simulink model "nonlinearAirframe"  (R2026a)
settings: Solver=ode3  StartTime=0  FixedStep=Ts  EnableMultiTasking=on
undefined symbols (not defined in the file): init, Vehicle
libraries: shared6dof x1, aerolibasang x1, dynamicsLibrary x1
settings Model: Creator=The MathWorks, Inc.  LastModifiedBy=khade
settings OptimizationCC: BufferReuse=off
settings DebuggingCC: ParameterPrecisionLossMsg=none
settings HardwareCC: ProdHWDeviceType=32-bit Generic

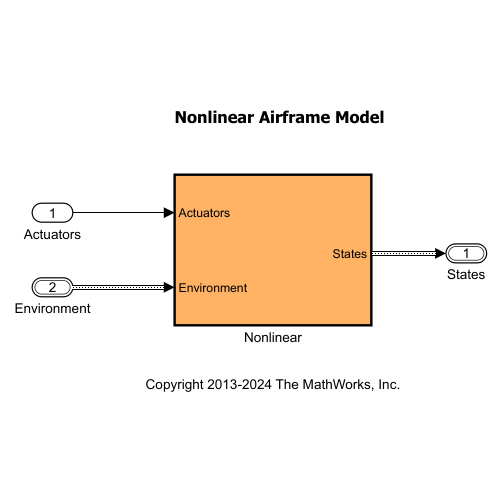
[thumbnail: Simulink's stored preview of the top-level diagram]
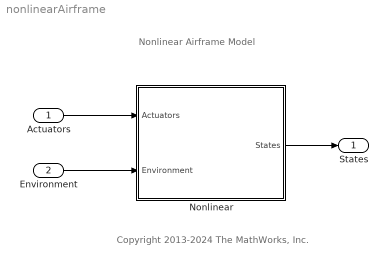
== system nonlinearAirframe ==
  note: Copyright 2013-2024 The MathWorks, Inc.
  note: Nonlinear Airframe Model
  Actuators : Inport  OutDataTypeStr=single  Unit=rpm  PortDimensions=[1 4]
  Environment : Inport  Port=2  OutDataTypeStr=Bus: EnvironmentBus  BusOutputAsStruct=on
  Nonlinear : Subsystem  TreatAsAtomicUnit=on
  States : Outport  OutDataTypeStr=Bus: StatesBus  VectorParamsAs1DForOutWhenUnconnected=off  BusOutputAsStruct=on
  wires:
  Actuators/1 -> Nonlinear/1(Actuators)
  Environment/1 -> Nonlinear/2(Environment)
  Nonlinear/1(States) -> States/1

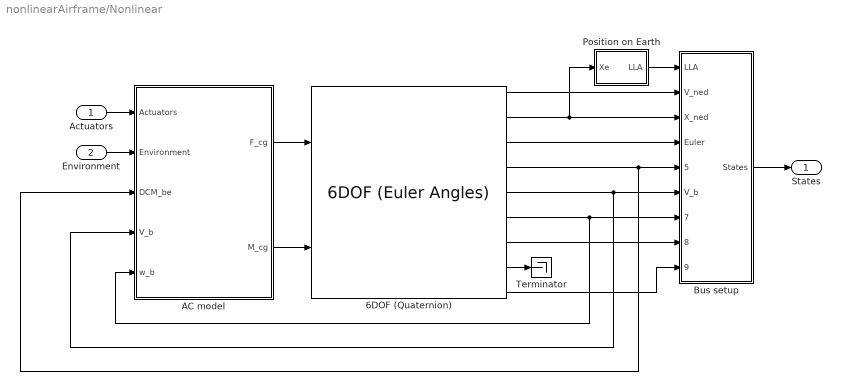
== system nonlinearAirframe/Nonlinear ==
  Actuators : Inport
  Environment : Inport  Port=2
  6DOF (Quaternion) : shared6dof/6DOF (Euler Angles)  units=Metric (MKS)  mtype=Fixed  rep=Euler Angles  xme_0=init.posNED  Vm_0=init.vb  eul_0=init.euler  pm_0=init.angRates  mass_0=Vehicle.Airframe.mass  mass_e=0.5  mass_f=2.0  inertia=Vehicle.Airframe.inertia  inertia_e=eye(3)  inertia_f=2*eye(3)  k_quat=Vehicle.SixDOF.quatGain  vre_flag=on  abi_flag=on  aMode=aMode  xme_statename=''  Vm_statename=''  eul_statename=''  quat_statename=''  pm_statename=''  mass_statename=''
  AC model : Subsystem
  Bus setup : Subsystem
  Position on Earth : Subsystem  Priority=1  TreatAsAtomicUnit=on
  Terminator : Terminator
  States : Outport  VectorParamsAs1DForOutWhenUnconnected=off
  wires:
  Actuators/1 -> AC model/1(Actuators)
  Environment/1 -> AC model/2(Environment)
  AC model/1(F_cg) -> 6DOF (Quaternion)/1
  AC model/2(M_cg) -> 6DOF (Quaternion)/2
  6DOF (Quaternion)/1 -> Bus setup/2(V_ned)
  6DOF (Quaternion)/2 -> Position on Earth/1(Xe), Bus setup/3(X_ned)
  6DOF (Quaternion)/3 -> Bus setup/4(Euler)
  6DOF (Quaternion)/6 -> AC model/5(w_b), Bus setup/7(Omega_b)
  6DOF (Quaternion)/7 -> Bus setup/8(dOmega_b)
  6DOF (Quaternion)/9 -> Bus setup/9(Accel_b)
  Bus setup/1(States) -> States/1
  Position on Earth/1(LLA) -> Bus setup/1(LLA)
  6DOF (Quaternion)/5 -> AC model/4(V_b), Bus setup/6(V_b)
  6DOF (Quaternion)/4 -> AC model/3(DCM_be), Bus setup/5(DCM_be)
  6DOF (Quaternion)/8 -> Terminator/1

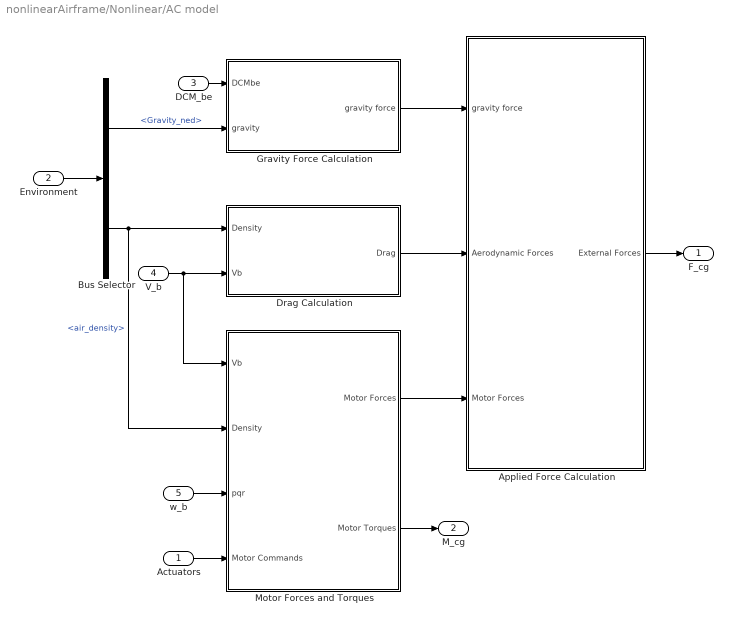
== system nonlinearAirframe/Nonlinear/AC model ==
  Actuators : Inport
  Environment : Inport  Port=2
  DCM_be : Inport  Port=3
  V_b : Inport  Port=4  Unit=m/s
  w_b : Inport  Port=5  Unit=rad/s
  Applied Force Calculation : Subsystem
  Bus Selector : BusSelector  OutputSignals=Gravity_ned,AtmosphereBus.air_density
  Drag Calculation : Subsystem
  Gravity Force Calculation : Subsystem
  Motor Forces and Torques : Subsystem
  F_cg : Outport  Unit=N  VectorParamsAs1DForOutWhenUnconnected=off
  M_cg : Outport  Port=2  Unit=N*m  VectorParamsAs1DForOutWhenUnconnected=off
  wires:
  Applied Force Calculation/1(External Forces) -> F_cg/1
  Motor Forces and Torques/2(Motor Torques) -> M_cg/1
  Motor Forces and Torques/1(Motor Forces) -> Applied Force Calculation/3(Motor Forces)
  Bus Selector/1 -> Gravity Force Calculation/2(gravity)  "<Gravity_ned>"
  Gravity Force Calculation/1(gravity force) -> Applied Force Calculation/1(gravity force)
  Environment/1 -> Bus Selector/1
  Bus Selector/2 -> Motor Forces and Torques/2(Density), Drag Calculation/1(Density)  "<air_density>"
  DCM_be/1 -> Gravity Force Calculation/1(DCMbe)
  V_b/1 -> Motor Forces and Torques/1(Vb), Drag Calculation/2(Vb)
  Drag Calculation/1(Drag) -> Applied Force Calculation/2(Aerodynamic Forces)
  Actuators/1 -> Motor Forces and Torques/4(Motor Commands)
  w_b/1 -> Motor Forces and Torques/3(pqr)

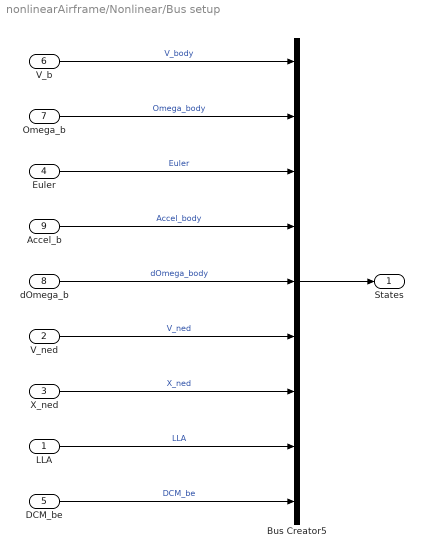
== system nonlinearAirframe/Nonlinear/Bus setup ==
  LLA : Inport  PortDimensions=3
  V_ned : Inport  Port=2  Unit=m/second  PortDimensions=3
  X_ned : Inport  Port=3  Unit=m  PortDimensions=3
  Euler : Inport  Port=4  Unit=rad  PortDimensions=3
  DCM_be : Inport  Port=5  PortDimensions=[3 3]
  V_b : Inport  Port=6  Unit=m/s  PortDimensions=3
  Omega_b : Inport  Port=7  Unit=rad/s  PortDimensions=3
  dOmega_b : Inport  Port=8  Unit=rad/s^2  PortDimensions=3
  Accel_b : Inport  Port=9  Unit=m/s^2  PortDimensions=3
  Bus Creator5 : BusCreator  Inputs=9  OutDataTypeStr=Bus: StatesBus  NonVirtualBus=on
  States : Outport  VectorParamsAs1DForOutWhenUnconnected=off
  wires:
  Bus Creator5/1 -> States/1
  V_b/1 -> Bus Creator5/1  "V_body"
  Omega_b/1 -> Bus Creator5/2  "Omega_body"
  Euler/1 -> Bus Creator5/3  "Euler"
  X_ned/1 -> Bus Creator5/7  "X_ned"
  Accel_b/1 -> Bus Creator5/4  "Accel_body"
  LLA/1 -> Bus Creator5/8  "LLA"
  dOmega_b/1 -> Bus Creator5/5  "dOmega_body"
  DCM_be/1 -> Bus Creator5/9  "DCM_be"
  V_ned/1 -> Bus Creator5/6  "V_ned"

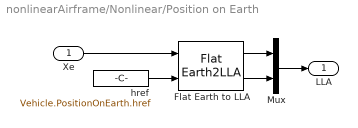
== system nonlinearAirframe/Nonlinear/Position on Earth ==
  Xe : Inport  Unit=m
  Flat Earth to LLA : FlatEarth2LLA  R=6378137  LL0=init.posLLA(1:2)  psi=Vehicle.PositionOnEarth.FlatEarthToLLA.xAxis
  Mux : Mux  Inputs=2
  href : Constant  Value=Vehicle.PositionOnEarth.href
  LLA : Outport  VectorParamsAs1DForOutWhenUnconnected=off
  wires:
  Mux/1 -> LLA/1
  Xe/1 -> Flat Earth to LLA/1
  Flat Earth to LLA/1 -> Mux/1
  Flat Earth to LLA/2 -> Mux/2
  href/1 -> Flat Earth to LLA/2

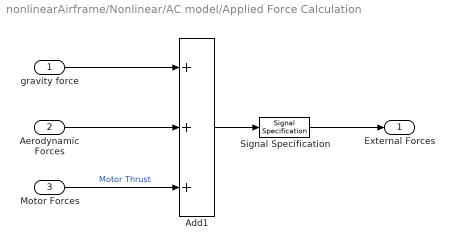
== system nonlinearAirframe/Nonlinear/AC model/Applied Force Calculation ==
  gravity force : Inport  Unit=N
  Aerodynamic Forces : Inport  Port=2  Unit=N
  Motor Forces : Inport  Port=3  Unit=N
  Add1 : Sum  Inputs=+++
  Signal Specification : SignalSpecification  Dimensions=3
  External Forces : Outport  Unit=N  VectorParamsAs1DForOutWhenUnconnected=off
  wires:
  Add1/1 -> Signal Specification/1
  Motor Forces/1 -> Add1/3  "Motor Thrust"
  Aerodynamic Forces/1 -> Add1/2
  gravity force/1 -> Add1/1
  Signal Specification/1 -> External Forces/1

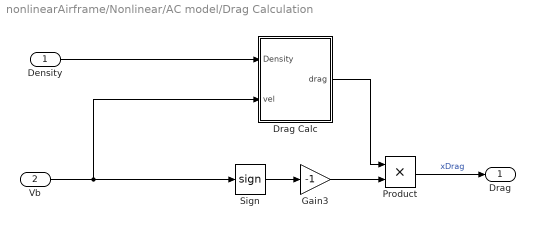
== system nonlinearAirframe/Nonlinear/AC model/Drag Calculation ==
  Density : Inport  Unit=kg/m^3
  Vb : Inport  Port=2  Unit=m/second
  Drag Calc : Subsystem
  Gain3 : Gain  Gain=-1
  Product : Product  RndMeth=Zero
  Sign : Signum  ZeroCross=off
  Drag : Outport  Unit=N  VectorParamsAs1DForOutWhenUnconnected=off
  wires:
  Density/1 -> Drag Calc/1(Density)
  Sign/1 -> Gain3/1
  Drag Calc/1(drag) -> Product/1
  Gain3/1 -> Product/2
  Product/1 -> Drag/1  "xDrag"
  Vb/1 -> Sign/1, Drag Calc/2(vel)

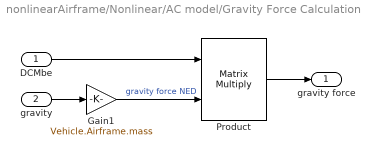
== system nonlinearAirframe/Nonlinear/AC model/Gravity Force Calculation ==
  DCMbe : Inport
  gravity : Inport  Port=2  Unit=m/s^2
  Gain1 : Gain  Gain=Vehicle.Airframe.mass
  Product : Product  Multiplication=Matrix(*)
  gravity force : Outport  Unit=N  VectorParamsAs1DForOutWhenUnconnected=off
  wires:
  gravity/1 -> Gain1/1
  Gain1/1 -> Product/2  "gravity force NED"
  Product/1 -> gravity force/1
  DCMbe/1 -> Product/1

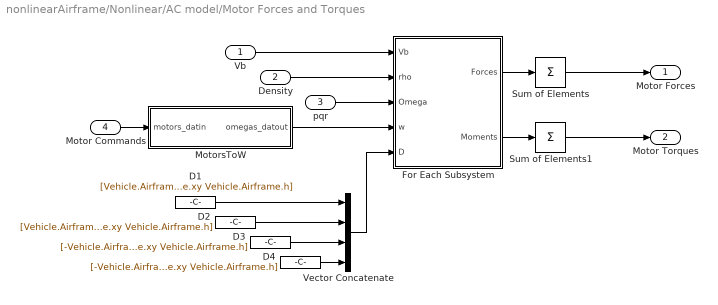
== system nonlinearAirframe/Nonlinear/AC model/Motor Forces and Torques ==
  Vb : Inport
  Density : Inport  Port=2
  pqr : Inport  Port=3
  Motor Commands : Inport  Port=4
  D1 : Constant  Value=[Vehicle.Airframe.xy -Vehicle.Airframe.xy Vehicle.Airframe.h]
  D2 : Constant  Value=[Vehicle.Airframe.xy Vehicle.Airframe.xy Vehicle.Airframe.h]
  D3 : Constant  Value=[-Vehicle.Airframe.xy Vehicle.Airframe.xy Vehicle.Airframe.h]
  D4 : Constant  Value=[-Vehicle.Airframe.xy -Vehicle.Airframe.xy Vehicle.Airframe.h]
  For Each Subsystem : Subsystem  TreatAsAtomicUnit=on
  MotorsToW : Subsystem
  Sum of Elements : Sum  Inputs=+  CollapseMode=Specified dimension  CollapseDim=2
  Sum of Elements1 : Sum  Inputs=+  CollapseMode=Specified dimension  CollapseDim=2
  Vector Concatenate : Concatenate  NumInputs=4  Mode=Multidimensional array  ConcatenateDimension=2
  Motor Forces : Outport  Unit=N  VectorParamsAs1DForOutWhenUnconnected=off
  Motor Torques : Outport  Port=2  Unit=N*m  VectorParamsAs1DForOutWhenUnconnected=off
  wires:
  D4/1 -> Vector Concatenate/4
  MotorsToW/1(omegas_datout) -> For Each Subsystem/4(w)
  Vector Concatenate/1 -> For Each Subsystem/5(D)
  For Each Subsystem/2(Moments) -> Sum of Elements1/1
  pqr/1 -> For Each Subsystem/3(Omega)
  Vb/1 -> For Each Subsystem/1(Vb)
  Motor Commands/1 -> MotorsToW/1(motors_datin)
  D1/1 -> Vector Concatenate/1
  D3/1 -> Vector Concatenate/3
  D2/1 -> Vector Concatenate/2
  Sum of Elements1/1 -> Motor Torques/1
  Density/1 -> For Each Subsystem/2(rho)
  Sum of Elements/1 -> Motor Forces/1
  For Each Subsystem/1(Forces) -> Sum of Elements/1

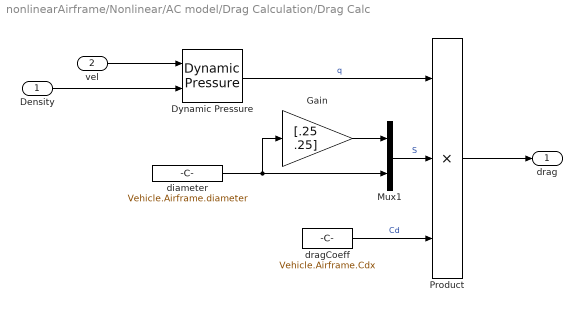
== system nonlinearAirframe/Nonlinear/AC model/Drag Calculation/Drag Calc ==
  Density : Inport  Unit=kg/m^3
  vel : Inport  Port=2  Unit=m/s
  Dynamic Pressure : aerolibasang/Dynamic Pressure
  Gain : Gain  Gain=[.25 .25]
  Mux1 : Mux  Inputs=2
  Product : Product  Inputs=3  RndMeth=Zero
  diameter : Constant  Value=Vehicle.Airframe.diameter  SampleTime=0
  dragCoeff : Constant  Value=Vehicle.Airframe.Cdx  SampleTime=0
  drag : Outport  Unit=N  VectorParamsAs1DForOutWhenUnconnected=off
  wires:
  Product/1 -> drag/1
  dragCoeff/1 -> Product/3  "Cd"
  Dynamic Pressure/1 -> Product/1  "q"
  diameter/1 -> Gain/1, Mux1/2
  Mux1/1 -> Product/2  "S"
  Gain/1 -> Mux1/1
  vel/1 -> Dynamic Pressure/1
  Density/1 -> Dynamic Pressure/2

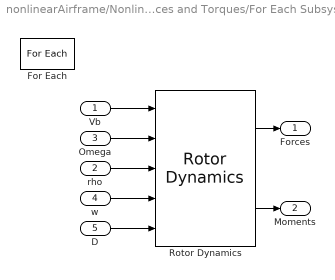
== system nonlinearAirframe/Nonlinear/AC model/Motor Forces and Torques/For Each Subsystem ==
  Vb : Inport  PortDimensions=3
  rho : Inport  Port=2  PortDimensions=1
  Omega : Inport  Port=3
  w : Inport  Port=4  Partition=on  PartitionDimension=2  PartitionWidth=1  PartitionOffset=0
  D : Inport  Port=5  Partition=on  PartitionDimension=2  PartitionWidth=1  PartitionOffset=0
  For Each : ForEach  DisableCoverage=on
  Rotor Dynamics : dynamicsLibrary/Rotor Dynamics  SystemSampleTime=-1  VariantActivationTime=update diagram  EmptyChoice=off  PassThrough=off  PassThroughVariantControl=(default)  EmptyChoiceVariantControl=(default)  AllowFlexibleInterface=on  Latency=0  AutoFrameSizeCalculation=off
      settings: SourceProductName=Aerospace Blockset
  Forces : Outport  ConcatenationDimension=2  VectorParamsAs1DForOutWhenUnconnected=off
  Moments : Outport  Port=2  ConcatenationDimension=2  VectorParamsAs1DForOutWhenUnconnected=off
  wires:
  Rotor Dynamics/1 -> Forces/1
  Rotor Dynamics/2 -> Moments/1
  Vb/1 -> Rotor Dynamics/1
  Omega/1 -> Rotor Dynamics/2
  rho/1 -> Rotor Dynamics/3
  D/1 -> Rotor Dynamics/5
  w/1 -> Rotor Dynamics/4

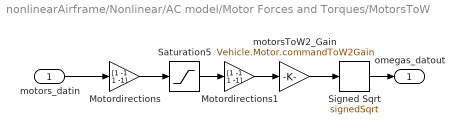
== system nonlinearAirframe/Nonlinear/AC model/Motor Forces and Torques/MotorsToW ==
  motors_datin : Inport
  Motordirections : Gain  Gain=[1 -1 1 -1]  ParamDataTypeStr=single  OutDataTypeStr=Inherit: Inherit via back propagation  SaturateOnIntegerOverflow=on
  Motordirections1 : Gain  Gain=[1 -1 1 -1]  ParamDataTypeStr=single  OutDataTypeStr=Inherit: Inherit via back propagation  SaturateOnIntegerOverflow=on
  Saturation5 : Saturate  UpperLimit=Vehicle.Motor.maxLimit  LowerLimit=Vehicle.Motor.minLimit  OutDataTypeStr=Inherit: Inherit via back propagation
  Signed Sqrt : Sqrt  Operator=signedSqrt  OutDataTypeStr=Inherit: Inherit via back propagation
  motorsToW2_Gain : Gain  Gain=Vehicle.Motor.commandToW2Gain  ParamDataTypeStr=single  OutDataTypeStr=Inherit: Inherit via back propagation  SaturateOnIntegerOverflow=on
  omegas_datout : Outport  VectorParamsAs1DForOutWhenUnconnected=off
  wires:
  motorsToW2_Gain/1 -> Signed Sqrt/1
  Motordirections/1 -> Saturation5/1
  Saturation5/1 -> Motordirections1/1
  Motordirections1/1 -> motorsToW2_Gain/1
  Signed Sqrt/1 -> omegas_datout/1
  motors_datin/1 -> Motordirections/1
